simulink model "electric_sim"  (R2023a)
settings: Solver=VariableStepAuto  StartTime=0.0  StopTime=10  RelTol=1e-3
libraries: fl_lib x12, nesl_utility x5
settings Model: Creator=ahmad  LastModifiedBy=ahmad

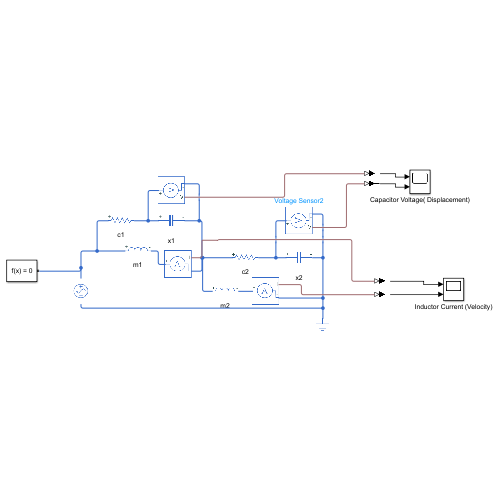
[thumbnail: Simulink's stored preview of the top-level diagram]
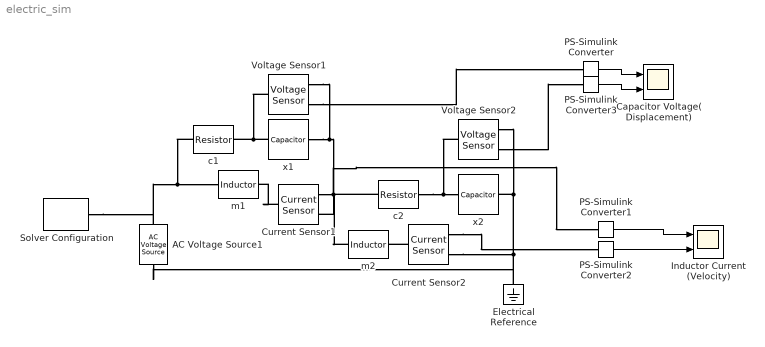
== system electric_sim ==
  AC Voltage Source1 : fl_lib/Electrical/Electrical Sources/AC Voltage Source  amp=5000 V  shift=0 deg  frequency=4 Hz  omega=0 rad/s
  Capacitor Voltage( Displacement) : Scope  NumInputPorts=2
  Current Sensor1 : fl_lib/Electrical/Electrical Sensors/Current Sensor
  Current Sensor2 : fl_lib/Electrical/Electrical Sensors/Current Sensor
  Electrical Reference : fl_lib/Electrical/Electrical Elements/Electrical Reference
  Inductor Current (Velocity) : Scope  NumInputPorts=2
  PS-Simulink Converter{,1..3} (4 alike) : nesl_utility/PS-Simulink Converter  PhysicalDomain=network_engine_domain  SubClassName=ps_output  LeftPortType=input  RightPortType=output  PseudoPeriodic=off  Frequencies=[]  VectorFormat=inherit  Unit=inherit  AffineConversion=off
  Solver Configuration : nesl_utility/Solver Configuration  PhysicalDomain=network_engine_domain  SubClassName=solver  LeftPortType=input  RightPortType=generic  Tones=[]  Harmonics=[]  SimulateNoise=off  Profile=off  UseLocalSampling=off  EnableSwitchedLinearOptims=on  FrequencyDomain=off  UseCCode=off  RelTol=0.001  AbsTol=0.001  MinStep=1e-09  ToWorkspace=off  RevertToSquareIcSolve=off  NumHomotopyIterations=100  PhasorMode=off  PhasorModeNumHarmonics=1  ConsistencySolver=NEWTON_XTOL_AFTER_FTOL  IndexReductionMethod=DerivativeReplacement  DoDC=off  ResidualTolerance=1e-09  ConsistencyTolSource=GLOBAL  ConsistencyAbsTol=0.001  ConsistencyRelTol=0.001  ConsistencyTolFactor=0.001  UseLocalSolver=off  LocalSolverChoice=NE_BACKWARD_EULER_ADVANCER  ResolveIndetEquations=on  FunctionEvalNumThread=1  LocalSolverSampleTime=0.001  DoFixedCost=off  MaxNonlinIter=3  MaxModeIter=2  ComputeImpulses=off  ImpulseIterations=2  LinearAlgebra=auto  LinearAlgebraNumThread=0  EquationFormulation=NE_TIME_EF  DelaysMemoryBudget=1024  AutomaticFiltering=on  FilteringTimeConstant=0.001  PartitionStorageMethod=AS_NEEDED  PartitionMemoryBudget=1024  PartitionMethod=ROBUST
  Voltage Sensor1 : fl_lib/Electrical/Electrical Sensors/Voltage Sensor
  Voltage Sensor2 : fl_lib/Electrical/Electrical Sensors/Voltage Sensor
  c1 : fl_lib/Electrical/Electrical Elements/Resistor  R=4 MOhm  i_specify=off  i_priority=None  i=0 A  i_nominal_specify=off  i_nominal_unit=A  i_nominal_value=1  v_specify=off  v_priority=None  v=0 V  v_nominal_specify=off  v_nominal_unit=V  v_nominal_value=1
  c2 : fl_lib/Electrical/Electrical Elements/Resistor  R=2 MOhm  i_specify=off  i_priority=None  i=0 A  i_nominal_specify=off  i_nominal_unit=A  i_nominal_value=1  v_specify=off  v_priority=None  v=0 V  v_nominal_specify=off  v_nominal_unit=V  v_nominal_value=1
  m1 : fl_lib/Electrical/Electrical Elements/Inductor  l=4000 H  r=0 Ohm  g=0 1/Ohm  i_specify=on  i_priority=None  i=0 A  i_nominal_specify=off  i_nominal_unit=A  i_nominal_value=1  v_specify=off  v_priority=None  v=0 V  v_nominal_specify=off  v_nominal_unit=V  v_nominal_value=1  i_L_specify=off  i_L_priority=High  i_L=0 A  i_L_nominal_specify=off  i_L_nominal_unit=A  i_L_nominal_value=1
  m2 : fl_lib/Electrical/Electrical Elements/Inductor  l=200 H  r=0 Ohm  g=0 1/Ohm  i_specify=on  i_priority=None  i=0 A  i_nominal_specify=off  i_nominal_unit=A  i_nominal_value=1  v_specify=off  v_priority=None  v=0 V  v_nominal_specify=off  v_nominal_unit=V  v_nominal_value=1  i_L_specify=off  i_L_priority=High  i_L=0 A  i_L_nominal_specify=off  i_L_nominal_unit=A  i_L_nominal_value=1
  x1 : fl_lib/Electrical/Electrical Elements/Capacitor  c=0.25 uF  r=0 Ohm  g=0 1/Ohm  i_specify=off  i_priority=None  i=0 A  i_nominal_specify=off  i_nominal_unit=A  i_nominal_value=1  v_specify=on  v_priority=None  v=0 V  v_nominal_specify=off  v_nominal_unit=V  v_nominal_value=1  vc_specify=off  vc_priority=High  vc=0 V  vc_nominal_specify=off  vc_nominal_unit=V  vc_nominal_value=1
  x2 : fl_lib/Electrical/Electrical Elements/Capacitor  c=5 uF  r=0 Ohm  g=0 1/Ohm  i_specify=off  i_priority=None  i=0 A  i_nominal_specify=off  i_nominal_unit=A  i_nominal_value=1  v_specify=on  v_priority=None  v=0 V  v_nominal_specify=off  v_nominal_unit=V  v_nominal_value=1  vc_specify=off  vc_priority=High  vc=0 V  vc_nominal_specify=off  vc_nominal_unit=V  vc_nominal_value=1
  wires:
  PS-Simulink Converter/1 -> Capacitor Voltage( Displacement)/1
  PS-Simulink Converter2/1 -> Inductor Current (Velocity)/2
  PS-Simulink Converter1/1 -> Inductor Current (Velocity)/1
  PS-Simulink Converter3/1 -> Capacitor Voltage( Displacement)/2
  connections:
  x1/LConn1 -- Voltage Sensor1/LConn1 -- c1/RConn1
  c1/LConn1 -- Solver Configuration/RConn1 -- AC Voltage Source1/LConn1 -- m1/LConn1
  Current Sensor1/LConn1 -- m1/RConn1
  x1/RConn1 -- Voltage Sensor1/RConn2 -- m2/LConn1 -- c2/LConn1 -- Current Sensor1/RConn2
  c2/RConn1 -- Voltage Sensor2/LConn1 -- x2/LConn1
  Current Sensor2/LConn1 -- m2/RConn1
  Current Sensor2/RConn2 -- AC Voltage Source1/RConn1 -- Electrical Reference/LConn1 -- Voltage Sensor2/RConn2 -- x2/RConn1
  Voltage Sensor1/RConn1 -- PS-Simulink Converter/LConn1
  Voltage Sensor2/RConn1 -- PS-Simulink Converter3/LConn1
  Current Sensor1/RConn1 -- PS-Simulink Converter1/LConn1
  Current Sensor2/RConn1 -- PS-Simulink Converter2/LConn1
